simulink model "fusion_sim"  (R2024b)
settings: Solver=FixedStepAuto  StartTime=0.0  StopTime=cfg.sim.T  FixedStep=cfg.sim.dt_imu  RelTol=1e-3
values from neighbouring files (symbols this model uses):
  cfg = struct()    [sim_config.m]    (also in sim_main.m = sim_config())
undefined symbols (not defined in the file or in its folder): fractalcoef, ins_x0
libraries: matrix_library x1, sensorgpslib x1, simulink_extras x1, mspsensorlib x1
settings Model: Creator=Mitchell  LastModifiedBy=Mitchell

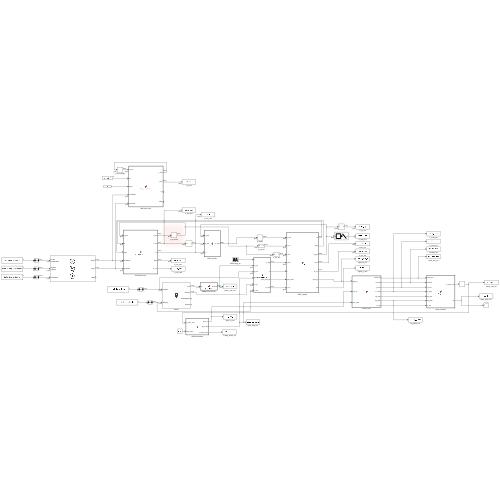
[thumbnail: Simulink's stored preview of the top-level diagram]
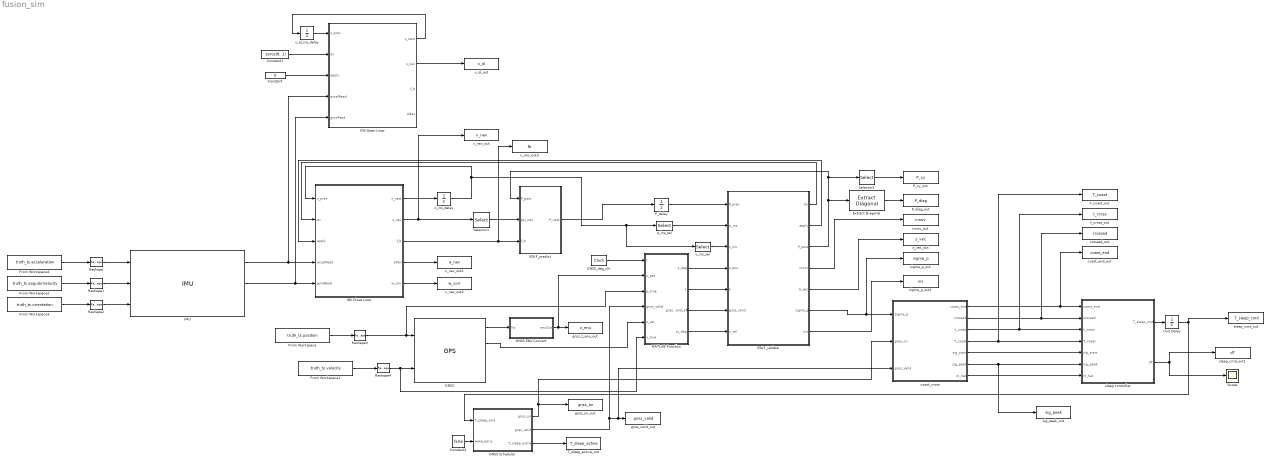
== system fusion_sim ==
  Constant : Constant  Value=0  OutDataTypeStr=boolean
  Constant1 : Constant  Value=zeros(8, 1)
  Constant2 : Constant  Value=false
  ESKF_predict : MATLAB Function  TreatAsAtomicUnit=on
  ESKF_update : MATLAB Function  TreatAsAtomicUnit=on
  Extract Diagonal : matrix_library/Extract Diagonal
      settings: LibrarySourceBlock=|
      | simulink/Matrix
      | Operations/Extract Diagonal
  From Workspace : FromWorkspace  VariableName=truth_ts.position  SampleTime=cfg.sim.dt_imu  Interpolate=off  OutputAfterFinalValue=Holding final value
  From Workspace1 : FromWorkspace  VariableName=truth_ts.velocity  OutDataTypeStr=double  SampleTime=cfg.sim.dt_imu  Interpolate=off  OutputAfterFinalValue=Holding final value
  From Workspace2 : FromWorkspace  VariableName=truth_ts.angularVelocity  SampleTime=cfg.sim.dt_imu  Interpolate=off  ZeroCross=off  OutputAfterFinalValue=Holding final value
  From Workspace3 : FromWorkspace  VariableName=truth_ts.orientation  SampleTime=cfg.sim.dt_imu  Interpolate=off  ZeroCross=off  OutputAfterFinalValue=Holding final value
  From Workspace4 : FromWorkspace  VariableName=truth_ts.acceleration  SampleTime=cfg.sim.dt_imu  Interpolate=off  ZeroCross=off  OutputAfterFinalValue=Holding final value
  GNSS : sensorgpslib/GPS  DispRefFrame=ENU  PositionInputFormat=Local  ReferenceLocation=cfg.gnss.ReferenceLocation  HorizontalPositionAccuracy=cfg.gnss.HorizontalPositionAccuracy  VerticalPositionAccuracy=cfg.gnss.VerticalPositionAccuracy  VelocityAccuracy=cfg.gnss.VelocityAccuracy  DecayFactor=cfg.gnss.DecayFactor  SeedDouble=cfg.gnss.Seed  SimulateUsing=Code generation
      settings: LibrarySourceBlock=mspsensorlib/GPS
  GNSS ENU Convert : MATLAB Function  TreatAsAtomicUnit=on
  GNSS Scheduler : MATLAB Function  TreatAsAtomicUnit=on
  GNSS_deg_clk : simulink_extras/Flip Flops/Clock  period=2
  IMU : mspsensorlib/IMU  DispRefFrame=ENU  TemperaturePort=off  Temperature=25  MagneticFieldPort=off  MagneticFieldNED=[ 27.5550, -2.4169, -16.0849 ]  MagneticFieldENU=[0, 0, 0]  SeedDouble=cfg.imu.Seed  SimulateUsing=Code generation  AccelParamsMeasurementRange=Inf  AccelParamsResolution=0  AccelParamsConstantBias=cfg.imu.accel.ConstantBias  AccelParamsAxesMisalignment=[ 100, 0, 0; 0, 100, 0; 0, 0, 100 ]  AccelParamsNoiseDensity=cfg.imu.accel.VelocityRandomWalk * [1 1 1]  AccelParamsBiasInstability=cfg.imu.accel.BiasInstability* [1 1 1]  AccelParamsBiasInstabilityNumerator=fractalcoef().Numerator  AccelParamsBiasInstabilityDenominator=fractalcoef().Denominator  AccelParamsRandomWalk=cfg.imu.accel.AccelerationRandomWalk * [1 1 1]  AccelParamsNoiseType=double-sided  AccelParamsTemperatureBias=[ 0, 0, 0 ]  AccelParamsTemperatureScaleFactor=[ 0, 0, 0 ]  GyroParamsMeasurementRange=Inf  GyroParamsResolution=0  GyroParamsConstantBias=cfg.imu.gyro.ConstantBias  GyroParamsAxesMisalignment=[ 100, 0, 0; 0, 100, 0; 0, 0, 100 ]  GyroParamsAccelerationBias=[ 0, 0, 0 ]  GyroParamsNoiseDensity=cfg.imu.gyro.AngleRandomWalk * [1 1 1]  GyroParamsBiasInstability=cfg.imu.gyro.BiasInstability * [1 1 1]  GyroParamsBiasInstabilityNumerator=fractalcoef().Numerator  GyroParamsBiasInstabilityDenominator=fractalcoef().Denominator  GyroParamsRandomWalk=cfg.imu.gyro.RateRandomWalk * [1 1 1]  GyroParamsNoiseType=double-sided  GyroParamsTemperatureBias=[ 0, 0, 0 ]  GyroParamsTemperatureScaleFactor=[ 0, 0, 0 ]  MagParamsMeasurementRange=Inf  MagParamsResolution=0  MagParamsConstantBias=[ 0, 0, 0 ]  MagParamsAxesMisalignment=[ 100, 0, 0; 0, 100, 0; 0, 0, 100 ]  MagParamsNoiseDensity=[ 0, 0, 0 ]  MagParamsBiasInstability=[ 0, 0, 0 ]  MagParamsBiasInstabilityNumerator=fractalcoef().Numerator  MagParamsBiasInstabilityDenominator=fractalcoef().Denominator  MagParamsRandomWalk=[ 0, 0, 0 ]  MagParamsNoiseType=double-sided  MagParamsTemperatureBias=[ 0, 0, 0 ]  MagParamsTemperatureScaleFactor=[ 0, 0, 0 ]
  INS Close Loop : MATLAB Function  TreatAsAtomicUnit=on  SystemSampleTime=cfg.sim.dt_imu
  INS Open Loop : MATLAB Function  TreatAsAtomicUnit=on  SystemSampleTime=cfg.sim.dt_imu
  MATLAB Function : MATLAB Function  TreatAsAtomicUnit=on
  P_delay : UnitDelay  InitialCondition=diag(cfg.eskf.P0_diag)  SampleTime=cfg.sim.dt_imu  HasFrameUpgradeWarning=on
  P_diag_out : ToWorkspace  VariableName=P_diag  SaveFormat=Timeseries  SampleTime=cfg.sim.dt_imu
  P_xy_out : ToWorkspace  VariableName=P_xy  SaveFormat=Timeseries  SampleTime=cfg.sim.dt_imu
  Reshape : Reshape  OutputDimensionality=Row vector (2-D)  OutputDimensions=[3,1]
  Reshape1 : Reshape  OutputDimensionality=Row vector (2-D)  OutputDimensions=[3,1]
  Reshape2 : Reshape  OutputDimensionality=Row vector (2-D)  OutputDimensions=[3,1]
  Reshape3 : Reshape  OutputDimensionality=Row vector (2-D)  OutputDimensions=[4,1]
  Reshape4 : Reshape  OutputDimensionality=Row vector (2-D)  OutputDimensions=[4,1]
  Scope : Scope
  Selector1 : Selector  InputPortWidth=8  IndexOptions=Index vector (dialog)  Indices=[5]  OutputSizes=1
  Selector2 : Selector  NumberOfDimensions=2  InputPortWidth=[8 8]  IndexOptions=Index vector (dialog),Index vector (dialog)  Indices=[1],[2]  OutputSizes=1,1
  T_coast_out : ToWorkspace  VariableName=T_coast  SaveFormat=Timeseries  SampleTime=-1
  T_sleep_active_out : ToWorkspace  VariableName=T_sleep_active  SaveFormat=Timeseries  SampleTime=-1
  Unit Delay : UnitDelay  InitialCondition=cfg.ctrl.T_sleep0  SampleTime=cfg.sim.dt_imu  HasFrameUpgradeWarning=on
  coast_cross : MATLAB Function  TreatAsAtomicUnit=on
  coast_end_out : ToWorkspace  VariableName=coast_end  SaveFormat=Timeseries  SampleTime=-1
  crossed_out : ToWorkspace  VariableName=crossed  SaveFormat=Timeseries  SampleTime=-1
  gnss_on_out : ToWorkspace  VariableName=gnss_on  SaveFormat=Timeseries  SampleTime=cfg.sim.dt_imu
  gnss_valid_out : ToWorkspace  VariableName=gnss_valid  SaveFormat=Timeseries  SampleTime=cfg.sim.dt_imu
  gnss_z_enu_out : ToWorkspace  VariableName=z_enu  SaveFormat=Timeseries  SampleTime=cfg.sim.dt_imu
  innov_out : ToWorkspace  VariableName=innov  SaveFormat=Timeseries  SampleTime=cfg.sim.dt_imu
  p_ins_sel : Selector  InputPortWidth=8  IndexOptions=Index vector (dialog)  Indices=[1 2]  OutputSizes=1
  s_vec_out : ToWorkspace  VariableName=s_vec  SaveFormat=Timeseries  SampleTime=cfg.sim.dt_imu
  sig_peak_out : ToWorkspace  VariableName=sig_peak  SaveFormat=Timeseries  SampleTime=-1
  sigma_p_out : ToWorkspace  VariableName=sigma_p  SaveFormat=Timeseries  SampleTime=cfg.sim.dt_imu
  sigma_p_out1 : ToWorkspace  VariableName=nis  SaveFormat=Timeseries  SampleTime=cfg.sim.dt_imu
  sleep controller : MATLAB Function  TreatAsAtomicUnit=on
  sleep_cmd_out : ToWorkspace  VariableName=T_sleep_cmd  SaveFormat=Timeseries  SampleTime=-1
  sleep_cmd_out1 : ToWorkspace  VariableName=dT  SaveFormat=Timeseries  SampleTime=-1
  t_cross_out : ToWorkspace  VariableName=t_cross  SaveFormat=Timeseries  SampleTime=-1
  v_ins_sel : Selector  InputPortWidth=8  IndexOptions=Index vector (dialog)  Indices=[3 4]  OutputSizes=1
  x_ins_delay : UnitDelay  InitialCondition=ins_x0 + cfg.ins.x0_err  SampleTime=cfg.sim.dt_imu  HasFrameUpgradeWarning=on
  x_nav_out : ToWorkspace  VariableName=x_nav  SaveFormat=Timeseries  SampleTime=cfg.sim.dt_imu
  x_nav_out1 : ToWorkspace  VariableName=a_nav  SaveFormat=Timeseries  SampleTime=cfg.sim.dt_imu
  x_nav_out2 : ToWorkspace  VariableName=w_corr  SaveFormat=Timeseries  SampleTime=cfg.sim.dt_imu
  x_nav_out3 : ToWorkspace  VariableName=fb  SaveFormat=Timeseries  SampleTime=cfg.sim.dt_imu
  x_ol_ins_delay : UnitDelay  InitialCondition=cfg.ins.x0  SampleTime=cfg.sim.dt_imu  HasFrameUpgradeWarning=on
  x_ol_out : ToWorkspace  VariableName=x_ol  SaveFormat=Timeseries  SampleTime=cfg.sim.dt_imu
  wires:
  From Workspace2/1 -> Reshape1/1
  From Workspace4/1 -> Reshape/1
  From Workspace1/1 -> Reshape4/1
  From Workspace/1 -> Reshape3/1
  GNSS/1 -> GNSS ENU Convert/1(lla)
  Reshape/1 -> IMU/1
  Reshape1/1 -> IMU/2
  From Workspace3/1 -> Reshape2/1
  Reshape3/1 -> MATLAB Function/3(p_true), GNSS/1
  Reshape4/1 -> MATLAB Function/6(v_true), GNSS/2
  Reshape2/1 -> IMU/3
  IMU/1 -> INS Open Loop/4(accelRead), INS Close Loop/4(accelRead)
  IMU/2 -> INS Open Loop/5(gyroRead), INS Close Loop/5(gyroRead)
  INS Close Loop/1(x_next) -> x_ins_delay/1
  INS Close Loop/2(x_nav) -> x_nav_out/1, Selector1/1
  Constant/1 -> INS Open Loop/3(apply)
  x_ol_ins_delay/1 -> INS Open Loop/1(x_prev)
  INS Open Loop/1(x_next) -> x_ol_ins_delay/1
  INS Open Loop/2(x_nav) -> x_ol_out/1
  Constant1/1 -> INS Open Loop/2(dx)
  ESKF_predict/1(P_next) -> P_delay/1
  P_delay/1 -> ESKF_update/1(P_prev)
  INS Close Loop/3(f_b) -> ESKF_predict/3(f_b), x_nav_out3/1
  ESKF_update/1(dx) -> INS Close Loop/2(dx)
  ESKF_update/3(P_post) -> ESKF_predict/1(P_post), Selector2/1, Extract Diagonal/1
  GNSS ENU Convert/1(enuOut) -> MATLAB Function/2(z_pos), gnss_z_enu_out/1
  GNSS Scheduler/2(gnss_valid) -> MATLAB Function/4(gnss_valid), coast_cross/3(gnss_valid), gnss_valid_out/1
  ESKF_update/2(apply) -> INS Close Loop/3(apply)
  x_ins_delay/1 -> INS Close Loop/1(x_prev), p_ins_sel/1, v_ins_sel/1
  Selector1/1 -> ESKF_predict/2(psi_nav)
  ESKF_update/5(S_vec) -> s_vec_out/1
  ESKF_update/4(innov) -> innov_out/1
  ESKF_update/6(sigma_p) -> coast_cross/1(sigma_p), sigma_p_out/1
  GNSS Scheduler/1(gnss_on) -> coast_cross/2(gnss_on), gnss_on_out/1
  Extract Diagonal/1 -> P_diag_out/1
  Selector2/1 -> P_xy_out/1
  p_ins_sel/1 -> ESKF_update/2(p_ins)
  INS Close Loop/4(aNav) -> x_nav_out1/1
  INS Close Loop/5(w_corr) -> x_nav_out2/1
  sleep controller/1(T_sleep_cmd) -> Unit Delay/1
  sleep controller/2(dT) -> sleep_cmd_out1/1, Scope/1
  Unit Delay/1 -> sleep_cmd_out/1, GNSS Scheduler/1(T_sleep_cmd)
  coast_cross/1(coast_end) -> coast_end_out/1, sleep controller/1(coast_end)
  coast_cross/2(crossed) -> crossed_out/1, sleep controller/2(crossed)
  coast_cross/3(t_cross) -> t_cross_out/1, sleep controller/3(t_cross)
  coast_cross/4(T_coast) -> T_coast_out/1, sleep controller/4(T_coast)
  coast_cross/6(sig_peak) -> sig_peak_out/1, sleep controller/6(sig_peak)
  Constant2/1 -> GNSS Scheduler/2(wake_early)
  GNSS Scheduler/3(T_sleep_active) -> T_sleep_active_out/1
  coast_cross/5(sig_start) -> sleep controller/5(sig_start)
  MATLAB Function/3(gnss_valid_eff) -> ESKF_update/6(gnss_valid)
  GNSS_deg_clk/1 -> MATLAB Function/1(t)
  MATLAB Function/1(z_deg) -> ESKF_update/4(z_enu)
  MATLAB Function/2(k) -> ESKF_update/5(k)
  v_ins_sel/1 -> ESKF_update/3(v_ins)
  GNSS/2 -> MATLAB Function/5(z_vel)
  MATLAB Function/4(zv_deg) -> ESKF_update/7(z_vel)
  coast_cross/7(m_hat) -> sleep controller/7(m_hat)
  ESKF_update/7(nis) -> sigma_p_out1/1

== matlab function fusion_sim/coast_cross ==
  data: coast_end output; crossed output; t_cross output; T_coast output; sig_start output; sigma_p input; gnss_on input boolean; gnss_valid input; sig_peak output; cross_prm parameter; m_hat output
function [coast_end, crossed, t_cross, T_coast, sig_start, sig_peak, m_hat] = ...
                                   coast_cross(sigma_p, gnss_on, gnss_valid, cross_prm)
%COAST_CROSS  Measures each coast: did sigma_p reach sigma_set, when, and
%                how fast was it growing?
%   A coast runs from receiver switch-off to the first valid fix after waking.
%   Its clock starts at 0 on the switch-off tick.
%     crossed   : sigma_p reached sigma_set during the coast
%     t_cross   : first time sigma_p >= sigma_set   [s]
%     T_coast   : time of the first fix             [s]
%     sig_start : sigma_p at switch-off             [m]
%     sig_peak  : highest sigma_p in the coast      [m]
%     m_hat     : measured growth exponent of D = sigma_p^2 - sig_start^2
%                 near the end of the coast, clamped to [2, 6].
%                 0 = no estimate (coast < 2 s or D not yet positive);
%                 sleep_ctrl then falls back to ctrl_prm.m_fix.
%   Outputs update on the coast_end tick and are held until the next one.
%
%   How m_hat is measured
%     sigma_p comes from P, which has no measurement noise in it, so two
%     points on the curve give the exponent exactly for that coast:
%         m_hat = ln(D_end / D_A) / ln(T_end / t_A)
%     The coast length is not known in advance, so D is sampled at doubling
%     checkpoints (1, 2, 4, 8, ... s) and the last two are kept. At the
%     end of the coast the older one (t_A) lies in [T_end/4, T_end/2), so
%     ln(T_end/t_A) >= ln 2 (well-conditioned) and the slope describes the
%     LATE part of the coast, which is the part being extrapolated.
%     Clamp [2, 6]: 2 = velocity-dominated growth, 6 = heading error through
%     f_b (gyro bias). Values outside that come from a stop's accel burst or
%     a cross-covariance transient, not a growth law to extrapolate from.
%#codegen
persistent was_on active k tx pk n_done cr_h tx_h Tc_h pk_h s0 s0_h
persistent tA DA tB DB tck m_h
if isempty(was_on)
    was_on = true;  active = false;  k = 0;  tx = -1;  pk = 0;  n_done = 0;
    cr_h = false;   tx_h = 0;  Tc_h = 0;  pk_h = 0; s0 = 0; s0_h = 0;
    tA = 0;  DA = 0;  tB = 0;  DB = 0;  tck = 1;  m_h = 0;
end
coast_end = false;

if was_on && ~gnss_on                 % receiver just switched off: coast starts
    active = true;  k = 0;  tx = -1;  pk = sigma_p;
    s0 = sigma_p;
    tA = 0;  DA = 0;  tB = 0;  DB = 0;  tck = 1;     % first checkpoint at 1 s
elseif active
    if gnss_valid                     % first fix: coast over
        active = false;  n_done = n_done + 1;
        cr_h = (tx >= 0);
        tx_h = max(tx, 0);
        Tc_h = (k + 1)*cross_prm.dt;        % this tick is k+1 ticks after switch-off
        pk_h = pk;
        s0_h = s0;

        % Growth exponent from the older checkpoint to the end of the coast
        D_end = pk^2 - s0^2;
        T_end = k*cross_prm.dt;             % last coast tick (pk includes it)
        if DA > 0 && D_end > DA && tA > 0
            m_h = log(D_end/DA) / log(T_end/tA);
            m_h = min(max(m_h, 2), 6);
        else
            m_h = 0;
        end

        coast_end = (n_done > cross_prm.n_skip);
    else
        k  = k + 1;
        pk = max(pk, sigma_p);
        if tx < 0 && sigma_p >= cross_prm.sigma_set
            tx = k*cross_prm.dt;            % first crossing of the target
        end
        if k*cross_prm.dt >= tck            % doubling checkpoint reached
            tA = tB;  DA = DB;
            tB = k*cross_prm.dt;  DB = sigma_p^2 - s0^2;
            tck = 2*tck;
        end
    end
end
was_on = gnss_on;

crossed = cr_h;  t_cross = tx_h;  T_coast = Tc_h;
sig_peak = pk_h; sig_start = s0_h; m_hat = m_h;

end

== matlab function fusion_sim/sleep controller ==
  data: coast_end input; crossed input; t_cross input; T_coast input; sig_start input; sig_peak input; m_hat input; T_sleep_cmd output; dT output; ctrl_prm parameter
function [T_sleep_cmd, dT] = sleep_ctrl(coast_end, crossed, t_cross, T_coast, ...
                                           sig_start, sig_peak, m_hat, ctrl_prm)
%SLEEP_CTRL  Updates the sleep length once per coast.
%   Error e = (ideal coast length) - (actual coast length):
%     Crossed     : e = t_cross - T_coast   (<= 0: the coast ran too long)
%     Not crossed : e = t_hat   - T_coast   (>= 0: room for a longer sleep)
%                   t_hat = T_coast * ((sigma_set^2 - sig_start^2)/D_end)^(1/m)
%   PI (adapt_en = true):  T = T_sleep0 + Kp*e + Ki*sum(e), clamped
%   Bang-bang (adapt_en = false): T = T -/+ dT_default, clamped (unchanged)
%
%   Changes from v1 (PI branch only; bang-bang baseline is untouched):
%   1. m from the data: m = m_hat (measured by coast_cross_v2) when
%      available, ctrl_prm.m_fix only as the fallback (m_hat = 0).
%   2. Sign of the proportional term: +Kp*e (v1 had -Kp*e, which pushed
%      against the integral term on every new error).
%   3. Anti-windup (conditional integration): the error is not added to
%      the integrator if that would push T further into a clamp it is
%      already against. Without it, a long outage (one coast of hundreds
%      of seconds -> large negative e) or a run of degraded coasts winds I
%      far negative, and T sits at T_min long after the fixes recover.
%   4. Unachievable coasts: if sig_start >= sigma_set, the fix itself was
%      already worse than the target (heavy degradation), so no sleep
%      length can meet it. T is commanded to T_min (keep sigma_p as low as
%      possible) but I is NOT updated, so when fixes recover the
%      controller returns to the sleep length it had learned before.
%#codegen
persistent T I dT_h
if isempty(T)
    T = ctrl_prm.T_sleep0; I = 0;  dT_h = 0;
end

if ctrl_prm.open_loop
    T = ctrl_prm.T_fix;
elseif coast_end
    T_prev = T;
    if ctrl_prm.adapt_en
        % ======== PI CONTROLLER ========
        if sig_start >= ctrl_prm.sigma_set
            % (4) target unachievable on this coast: be cautious, don't learn
            T = ctrl_prm.T_min;
        else
            if crossed
                e = t_cross - T_coast;
            else
                % (1) growth exponent: measured if available, else fixed
                m = ctrl_prm.m_fix;
                if m_hat > 0
                    m = m_hat;
                end
                D_end = sig_peak^2 - sig_start^2;
                if D_end > 0
                    t_hat = T_coast * ((ctrl_prm.sigma_set^2 - sig_start^2) ...
                                       / D_end)^(1/m);
                    e = t_hat - T_coast;
                else
                    e = 0;
                end
            end

            % (3) conditional integration: skip if it deepens saturation
            T_try  = ctrl_prm.T_sleep0 + ctrl_prm.Kp*e + ctrl_prm.Ki*(I + e);
            windup = (T_try > ctrl_prm.T_max && e > 0) || ...
                     (T_try < ctrl_prm.T_min && e < 0);
            if ~windup
                I = I + e;
            end

            % (2) correct sign on the proportional term
            T_raw = ctrl_prm.T_sleep0 + ctrl_prm.Kp*e + ctrl_prm.Ki*I;
            T = min(max(T_raw, ctrl_prm.T_min), ctrl_prm.T_max);
        end
    else
        % ======== BANG-bang Baseline (unchanged) ========
        if crossed
            T = T - ctrl_prm.dT_default;
        else
            T = T + ctrl_prm.dT_default;
        end
        T = min(max(T, ctrl_prm.T_min), ctrl_prm.T_max);
    end
    dT_h = T - T_prev;
end

T_sleep_cmd = T;  dT = dT_h;
end

== matlab function fusion_sim/MATLAB Function ==
  data: t input; z_deg output; z_pos input; p_true input; gnss_valid input; z_vel input; v_true input; k output; gnss_valid_eff output boolean; deg_prm parameter; zv_deg output
function [z_deg, k, gnss_valid_eff, zv_deg] = ...
            gnss_degrade(t, z_pos, p_true, gnss_valid, z_vel, v_true, deg_prm)
%GNSS_DEGRADE  Time-scheduled GNSS degradation, position AND velocity.
%
%     z_deg  = p_true + k*(z_pos - p_true)     position error std grows by k
%     zv_deg = v_true + k*(z_vel - v_true)     velocity error std grows by k
%     k      -> ESKF: BOTH position and velocity R are scaled by k^2
%     gnss_valid_eff = gnss_valid AND (k < k_out)   outage drops both
%
%   Why the same k for velocity: the degraded environments modelled here
%   (canopy / urban canyon) degrade the whole fix - fewer satellites,
%   worse geometry (DOP) and multipath affect Doppler velocity as well as
%   pseudorange position. Doppler usually degrades somewhat less, so a
%   shared k is a slightly conservative (pessimistic) choice. It also needs
%   NO new deg_prm fields, so build_sim_params.m is unchanged for this block.
%   Because R is scaled by the same k, the filter stays consistent with the
%   error actually injected.
%
%   Inputs
%     t          : simulation time (Clock block)                     [s]
%     z_pos      : GNSS position in the local ENU frame              [m]
%     p_true     : truth position (3D padding fine)                  [m]
%     gnss_valid : fix-available pulse from gnss_schedule
%     z_vel      : GPS block Velocity output, local ENU (1x3)        [m/s]
%                  (GPS block 'Reference frame' must be ENU - if NED,
%                   the first two elements are [vN vE], not [vE vN])
%     v_true     : truth velocity, same frame (truth.velocity)       [m/s]
%     deg_prm    : flat struct from build_sim_params (Parameter scope)
%                  en (0/1), t (1xN segment starts), k (1xN), k_out
%
%   Outputs
%     z_deg, k, gnss_valid_eff
%     zv_deg     : (2x1) degraded horizontal GNSS velocity [vE; vN]  [m/s]
%
%   With deg_prm.en = 0: z_deg = z_pos, zv_deg = z_vel(1:2), k = 1.
%#codegen

% Position: truth reshaped to the size of z_pos (fixed size on every path)
p = reshape(p_true(1:numel(z_pos)), size(z_pos));

% Velocity: horizontal channel only, always a 2x1 column for the ESKF
zv = reshape(z_vel(1:2),  2, 1);
vt = reshape(v_true(1:2), 2, 1);

k = 1;
if deg_prm.en ~= 0
    % Piecewise-constant lookup: k of the last segment that has started
    for i = 1:numel(deg_prm.t)
        if t >= deg_prm.t(i)
            k = deg_prm.k(i);
        end
    end
end

z_deg  = p  + k*(z_pos - p);       % k = 1 -> exact pass-through
zv_deg = vt + k*(zv - vt);
gnss_valid_eff = logical(gnss_valid) && (k < deg_prm.k_out);
end

== matlab function fusion_sim/INS Close Loop ==
  data: x_prev input size=[8 1]; dx input size=[8 1]; apply input boolean size=1; accelRead input; gyroRead input; x_next output size=[8 1]; x_nav output size=[8 1]; f_b output size=[2 1]; aNav output size=[2 1]; ins_prm parameter; w_corr output
function [x_next, x_nav, f_b, aNav, w_corr] = ins_mechanise(x_prev, dx, apply, ...
                                                    accelRead, gyroRead, ins_prm)
%INS_MECHANISE Correct-then-propagate strapdown mechanisation (2D, ENU).
%
%   x = [pE pN vE vN psi b_ax b_ay b_gz]'
%
%   x_prev     (8x1)  state from the Unit Delay
%   dx         (8x1)  correction from the ESKF
%   apply      (1x1)  true on update ticks
%   accelRead  (1x3)  raw accelerometer, body [m/s^2]
%   gyroRead   (1x3)  raw gyro, body [rad/s]
%   ins_prm               dt, accelInv, feedback
%
%   x_next     (8x1)  -> Unit Delay
%   x_nav      (8x1)  navigation output at THIS instant (log this)
%   f_b        (2x1)  bias-corrected specific force -> ESKF
%   aNav       (2x1)  nav-frame acceleration
%#codegen

    x = x_prev;

    %% 1. Correct
    if apply && ins_prm.feedback
        x    = x + dx;
        x(5) = wrap2pi(x(5));
    end
    x_nav = x;                       % output BEFORE propagating: refers to t_k

    %% 2. Propagate
    p   = x(1:2);
    v   = x(3:4);
    psi = x(5);
    b_a = x(6:7);
    b_g = x(8);

    a_meas = reshape(accelRead(1:2), 2, 1);       % force column, whatever the bus gives
    f_b    = ins_prm.accelInv * a_meas - b_a;

    c = cos(psi);
    s = sin(psi);
    aNav = [c, -s; s, c] * f_b;                   % body -> nav

    p_n   = p + v*ins_prm.dt + 0.5*aNav*ins_prm.dt^2;
    v_n   = v + aNav*ins_prm.dt;
    psi_n = wrap2pi(psi + (gyroRead(3) - b_g)*ins_prm.dt);

    w_corr = gyroRead(3) - b_g;      % 1x1

    x_next = [p_n; v_n; psi_n; b_a; b_g];
end

== matlab function fusion_sim/GNSS ENU Convert ==
  data: lla input; enuOut output
function enuOut = lla_2_ENU(lla)
%% ENUCONVERSION Converts LAT,LONG,ALTITUDE to ENU frame

lla_convert = lla2enu(lla, [0, 0, 0], "flat");
enuOut = lla_convert(1:2)';

end

== matlab function fusion_sim/GNSS Scheduler ==
  data: gnss_on output; T_sleep_cmd input; wake_early input; gnss_valid output boolean; T_sleep_active output double; sched_prm parameter
function [gnss_on, gnss_valid, T_sleep_active] = gnss_schedule(T_sleep_cmd, wake_early, sched_prm)
%GNSS_SCHEDULE  Receiver state machine: WARMUP -> ACTIVE -> SLEEP -> REACQ -> ACTIVE ...
%   gnss_on    : receiver powered (energy / duty cycle)
%   gnss_valid : one-tick pulse per fix at f_gnss (drives the ESKF update)
%   T_sleep_cmd is latched only on entry to SLEEP.
%#codegen
persistent mode k n_fix T_lat
WARMUP = uint8(0); ACTIVE = uint8(1); SLEEP = uint8(2); REACQ = uint8(3);
if isempty(mode)
    mode = WARMUP; k = 0; n_fix = 0; T_lat = sched_prm.T_sleep0;
end

k_fix   = round(1/(sched_prm.f_gnss*sched_prm.dt));   % ticks between fixes
N_fix   = round(sched_prm.T_active*sched_prm.f_gnss); % fixes per active window
k_warm  = round(sched_prm.T_warmup/sched_prm.dt);
k_reacq = round(sched_prm.t_reacq/sched_prm.dt);

gnss_valid = false;
switch mode
    case WARMUP
        gnss_on    = true;
        gnss_valid = (mod(k, k_fix) == 0);
        k = k + 1;
        if k >= k_warm
            mode = ACTIVE; k = 0; n_fix = 0;
        end
    case ACTIVE
        gnss_on    = true;
        gnss_valid = (mod(k, k_fix) == 0);  % first fix on the first ACTIVE tick
        k = k + 1;
        if gnss_valid, n_fix = n_fix + 1; end
        if n_fix >= N_fix
            mode  = SLEEP; k = 0;
            T_lat = T_sleep_cmd;            % latch at the falling edge
        end
    case SLEEP
        gnss_on = false;
        k = k + 1;
        if k >= round(T_lat/sched_prm.dt) || wake_early
            mode = REACQ; k = 0;
        end
    otherwise   % REACQ: powered, acquiring, no fix yet
        gnss_on = true;
        k = k + 1;
        if k >= k_reacq
            mode = ACTIVE; k = 0; n_fix = 0;
        end
end
T_sleep_active = T_lat;
end

== matlab function fusion_sim/ESKF_update ==
  data: P_prev input size=[8 8]; dx output size=[8 1]; p_ins input size=[2 1]; v_ins input; z_enu input size=[2 1]; k input; gnss_valid input boolean size=1; z_vel input; apply output boolean size=1; P_post output size=[8 8]; innov output size=[2 1]; S_vec output size=[3 1]; sigma_p output size=1; eskf_prm parameter; nis output
function [dx, apply, P_post, innov, S_vec, sigma_p, nis] = ...
            eskf_update(P_prev, p_ins, v_ins, z_enu, k, gnss_valid, z_vel, eskf_prm)
%ESKF_UPDATE LC error-state KF update with GNSS position + velocity.
%
%   z = [z_pos; z_vel],   y = z - [p_ins; v_ins],   H = [I2 0 0; 0 I2 0]
%
%   P_prev      (8x8)   Covariance predicted to this tick
%   p_ins       (2x1)   INS position, delayed state x_k-  (x_prev(1:2))
%   z_enu       (2x1)   GNSS position fix, ENU [m]
%   k           (1x1)   Degradation multiplier (scales R)
%   gnss_valid  (1x1)   True on exactly one tick per fix
%   v_ins       (2x1)   INS velocity, delayed state x_k-  (x_prev(3:4))
%   z_vel       (2x1)   GNSS velocity fix, ENU [m/s]
%   eskf_prm            R_sigma, Rv_sigma
%
%#codegen

    P = 0.5*(P_prev + P_prev.');

    dx    = zeros(8,1);
    apply = false;
    innov = zeros(2,1);
    S_vec = zeros(3,1);
    nis   = 0;

    if gnss_valid
        H  = [eye(2),     zeros(2,6);
              zeros(2,2), eye(2), zeros(2,4)];                  % 4x8
        Rm = k^2 * blkdiag(eskf_prm.R_sigma^2  * eye(2), ...
                           eskf_prm.Rv_sigma^2 * eye(2));       % 4x4

        y = [reshape(z_enu(1:2), 2, 1) - reshape(p_ins(1:2), 2, 1);
             reshape(z_vel(1:2), 2, 1) - reshape(v_ins(1:2), 2, 1)];   % 4x1
        S = H*P*H.' + Rm;        % 4x4
        K = (P*H.') / S;         % 8x4
        dx = K*y;
        nis = y.' * (S \ y);     % 4-dof NIS

        IKH = eye(8) - K*H;
        P   = IKH*P*IKH.' + K*Rm*K.';      % Joseph form
        P   = 0.5*(P + P.');

        apply = true;
        innov = y(1:2);
        S_vec = [S(1,1); S(2,2); S(1,2)];
    end

    P_post  = P;
    sigma_p = sqrt(max(P(1,1) + P(2,2), 0));
end

== matlab function fusion_sim/INS Open Loop ==
  data: x_prev input size=[8 1]; dx input size=[8 1]; apply input boolean size=1; accelRead input; gyroRead input; x_next output size=[8 1]; x_nav output size=[8 1]; f_b output size=[2 1]; aNav output size=[2 1]; ins_prm parameter
function [x_next, x_nav, f_b, aNav] = ins_mechanise(x_prev, dx, apply, ...
                                                    accelRead, gyroRead, ins_prm)
%INS_MECHANISE Correct-then-propagate strapdown mechanisation (2D, ENU).
%
%   x = [pE pN vE vN psi b_ax b_ay b_gz]'
%
%   x_prev     (8x1)  state from the Unit Delay
%   dx         (8x1)  correction from the ESKF
%   apply      (1x1)  true on update ticks
%   accelRead  (1x3)  raw accelerometer, body [m/s^2]
%   gyroRead   (1x3)  raw gyro, body [rad/s]
%   ins_prm               dt, accelInv, feedback
%
%   x_next     (8x1)  -> Unit Delay
%   x_nav      (8x1)  navigation output at THIS instant (log this)
%   f_b        (2x1)  bias-corrected specific force -> ESKF
%   aNav       (2x1)  nav-frame acceleration
%#codegen

    x = x_prev;

    %% 1. Correct
    if apply && ins_prm.feedback
        x    = x + dx;
        x(5) = wrap2pi(x(5));
    end
    x_nav = x;                       % output BEFORE propagating: refers to t_k

    %% 2. Propagate
    p   = x(1:2);
    v   = x(3:4);
    psi = x(5);
    b_a = x(6:7);
    b_g = x(8);

    a_meas = reshape(accelRead(1:2), 2, 1);       % force column, whatever the bus gives
    f_b    = ins_prm.accelInv * a_meas - b_a;

    c = cos(psi);
    s = sin(psi);
    aNav = [c, -s; s, c] * f_b;                   % body -> nav

    p_n   = p + v*ins_prm.dt + 0.5*aNav*ins_prm.dt^2;
    v_n   = v + aNav*ins_prm.dt;
    psi_n = wrap2pi(psi + (gyroRead(3) - b_g)*ins_prm.dt);

    x_next = [p_n; v_n; psi_n; b_a; b_g];
end

== matlab function fusion_sim/ESKF_predict ==
  data: P_post input size=[8 8]; P_next output size=[8 8]; psi_nav input size=1; f_b input size=[2 1]; eskf_prm parameter
function P_next = eskf_predict(P_post, psi_nav, f_b, eskf_prm)
%ESKF_PREDICT Covariance prediction for the error-state KF.
%
%   P_post   (8x8)  covariance after this tick's update
%   psi_nav  (1x1)  CORRECTED INS heading at this tick [rad]
%   f_b      (2x1)  bias-corrected specific force, body frame [m/s^2]
%   eskf_prm        dt, Na, Ng, Ka, Kg, Q_scale
%
%   P_next   (8x8)  covariance predicted to the next tick -> Unit Delay
%#codegen

    dt = eskf_prm.dt;
    c  = cos(psi_nav);
    s  = sin(psi_nav);

    Rbn   = [ c, -s;  s,  c];      % body -> nav,  R(psi)
    Rbn90 = [-s, -c;  c, -s];      % dR/dpsi     = R(psi + pi/2)

    A = zeros(8,8);
    A(1:2,3:4) = eye(2);           % d(dp)/dt = dv
    A(3:4,5)   = Rbn90 * f_b;      % heading error -> velocity error
    A(3:4,6:7) = -Rbn;             % accel bias    -> velocity error
    A(5,8)     = -1;               % gyro bias     -> heading error

    Adt = A*dt;
    F   = eye(8) + Adt + 0.5*(Adt*Adt);

    G = zeros(8,6);
    G(3:4,1:2) = -Rbn;             % accel white noise
    G(5,3)     = -1;               % gyro white noise
    G(6:7,4:5) = eye(2);           % accel bias random walk
    G(8,6)     = 1;                % gyro bias random walk

    Qc = diag([eskf_prm.Na^2, eskf_prm.Na^2, eskf_prm.Ng^2, ...
               eskf_prm.Ka^2, eskf_prm.Ka^2, eskf_prm.Kg^2]) * eskf_prm.Q_scale;

    M  = G*Qc*G.';
    Qd = 0.5*(F*M*F.' + M) * dt;   % trapezoidal (van Loan) discretisation

    P_next = F*P_post*F.' + Qd;
    P_next = 0.5*(P_next + P_next.');
end
